simulink model "surrogate_model_16"  (R2026a)
settings: Solver=VariableStepAuto
settings Model: Creator=shuki  LastModifiedBy=shuki

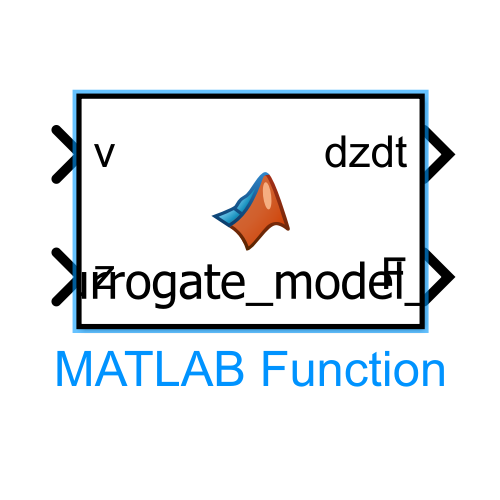
[thumbnail: Simulink's stored preview of the top-level diagram]
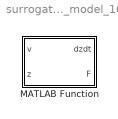
== system surrogate_model_16 ==
  MATLAB Function : MATLAB Function  TreatAsAtomicUnit=on

== matlab function surrogate_model_16/MATLAB Function ==
  data: dzdt output; F output; v input; z input
function [dzdt, F] = surrogate_model_16(v, z)

    S0 = 10^5;
    C1 = 32.762203;
    C2 = 55.41855;

    dzdt = v - ( abs(S0*C1*v) + (S0*v)^2 )*( z / (abs(S0*v) + C2) );

    F = 10^5 * z + 316.2277 * dzdt + 0.4 * v;

end
